simulink model "S_Tek_NDI_6DOF"  (R2025b)
settings: Solver=ode4  StartTime=0.0  StopTime=5  FixedStep=0.001  RelTol=1e-3
undefined symbols (not defined in the file): X, Y, Z
libraries: sm_lib x15, nesl_utility x13, instrumentseriallib x3, svdutilitieslib x2, sharedtransform x1, aerolibanimutils x1
(part 1 of 2)
settings Model: SimulationMode=accelerator  Creator=serha  LastModifiedBy=serha
settings OptimizationCC: DefaultParameterBehavior=Inlined  EnhancedBackFolding=on  PassReuseOutputArgsAs=Individual arguments  ZeroExternalMemoryAtStartup=off  ZeroInternalMemoryAtStartup=off  OptimizeBlockOrder=speed  DifferentSizesBufferReuse=on  EfficientTunableParamExpr=on
settings DebuggingCC: ParameterTunabilityLossMsg=error
settings SFSimCC: MATLABDynamicMemAlloc=off
settings RTWCC: SystemTargetFile=ert.tlc  GenCodeOnly=on  TemplateMakefile=ert_default_tmf  TargetLang=C++  Description=Embedded Coder
settings CodeAppCC: ForceParamTrailComments=on  IgnoreCustomStorageClasses=off  OperatorAnnotations=on  SimulinkDataObjDesc=on  SFDataObjDesc=on  InsertBlockDesc=on
settings ERTTargetCC: RootIOFormat=Structure reference  ERTCustomFileTemplate=example_file_process.tlc  TargetLangStandard=C++11 (ISO)  GenerateSampleERTMain=on  CodeInterfacePackaging=C++ class  SubcomponentCodeInterfacePackaging=C++ class

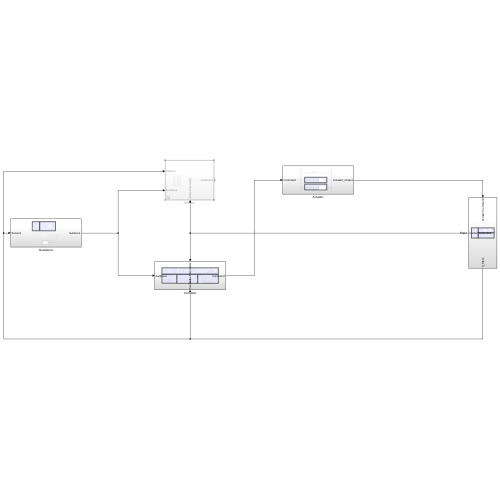
[thumbnail: Simulink's stored preview of the top-level diagram]
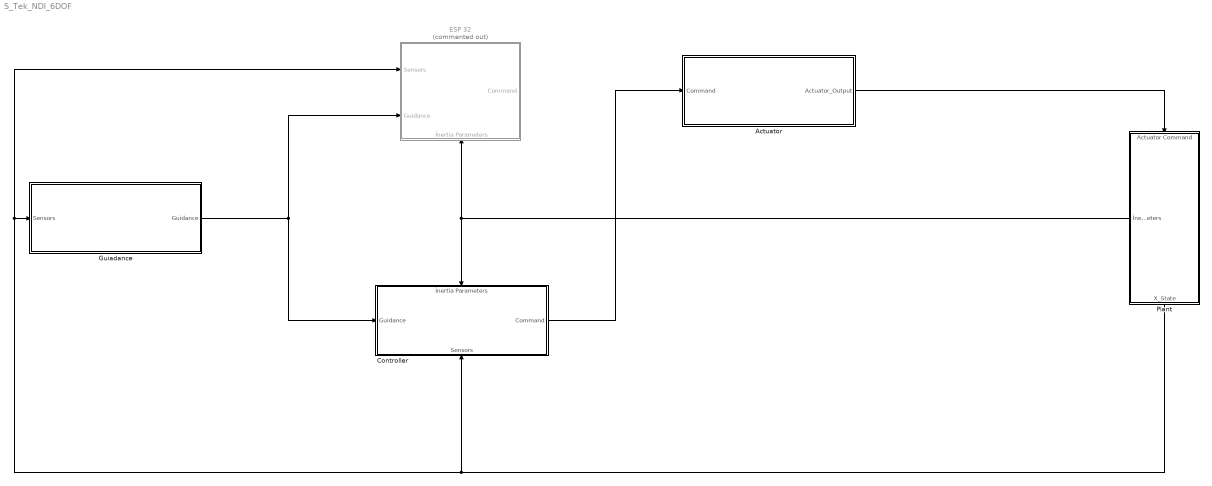
== system S_Tek_NDI_6DOF ==
  Actuator : Subsystem
  Controller : Subsystem
      settings: PortSchema="{\"entries\":[{\"content\":{\"sides\":[{\"content\":{\"connectorIds\":[\"In1\"]},\"type\":\"ConnectorPlacement.EquallySpacedRectSide\",\"uuid\":\"33b79308-0fc5-4fde-badb-0b37289253ef\"},{\"content\":{\"connectorIds\":[\"Out1\"],\"side\":\"RIGHT\"},\"type\":\"ConnectorPlacement.EquallySpacedRectSide\",\"uuid\":\"6727f24a-0c3c-4ca7-b1aa-847be9f11281\"},{\"content\":{\"connectorIds\":[\"In2\"],\"side\":\"TOP\"},\"type\":\"ConnectorPlacement.EquallySpacedRectSide\",\"uuid\":\"ebfc38b6-8c70-4d5f-9489-ae3a6562aa2e\"},{\"content\":{\"connectorIds\":[\"In3\"],\"side\":\"BOTTOM\"},\"type\":\"ConnectorPlacement.EquallySpacedRectSide\",\"uuid\":\"1b890ac9-3b95-4a4a-b282-16e3ecaf3aa4\"}]},\"type\":\"ConnectorPlacement.EquallySpacedConnector\",\"uuid\":\"d0cee92c-e3ff-4de0-b538-2dada08257b1\"}],\"packageUris\":[\"http://schema.mathworks.com/mf0/Connector/R2020b\"],\"version\":\"1.0\"}"
  ESP 32 : Subsystem  Commented=on
      settings: PortSchema="{\"entries\":[{\"content\":{\"sides\":[{\"content\":{\"connectorIds\":[\"In1\",\"In2\"]},\"type\":\"ConnectorPlacement.EquallySpacedRectSide\",\"uuid\":\"b68df156-6ec7-4598-b026-4cab0d4d3268\"},{\"content\":{\"connectorIds\":[\"Out1\"],\"side\":\"RIGHT\"},\"type\":\"ConnectorPlacement.EquallySpacedRectSide\",\"uuid\":\"75bb1db0-dca3-4be2-aa03-0ad52a7325c4\"},{\"content\":{\"side\":\"TOP\"},\"type\":\"ConnectorPlacement.EquallySpacedRectSide\",\"uuid\":\"cbcd1633-6d11-4a93-ac28-ed36ff8afac7\"},{\"content\":{\"connectorIds\":[\"In3\"],\"side\":\"BOTTOM\"},\"type\":\"ConnectorPlacement.EquallySpacedRectSide\",\"uuid\":\"f395c96f-7e1a-4722-a710-beafc27741bb\"}]},\"type\":\"ConnectorPlacement.EquallySpacedConnector\",\"uuid\":\"ea343adf-7795-4ee6-84a9-2bc60d61a1c3\"}],\"packageUris\":[\"http://schema.mathworks.com/mf0/Connector/R2020b\"],\"version\":\"1.0\"}"
  Guiadance : Subsystem
  Plant : Subsystem
      settings: PortSchema="{\"entries\":[{\"content\":{\"sides\":[{\"content\":{\"connectorIds\":[\"In1\"]},\"type\":\"ConnectorPlacement.EquallySpacedRectSide\",\"uuid\":\"29c8d766-87fc-4873-bda8-7cdfe26d04f7\"},{\"content\":{\"connectorIds\":[\"Out1\"],\"side\":\"RIGHT\"},\"type\":\"ConnectorPlacement.EquallySpacedRectSide\",\"uuid\":\"1efea905-e967-45fe-8852-2a4bff90dd9a\"},{\"content\":{\"side\":\"TOP\"},\"type\":\"ConnectorPlacement.EquallySpacedRectSide\",\"uuid\":\"b263cb17-9e53-4a4f-8000-fee4e63dac0a\"},{\"content\":{\"connectorIds\":[\"Out2\"],\"side\":\"BOTTOM\"},\"type\":\"ConnectorPlacement.EquallySpacedRectSide\",\"uuid\":\"2ade8f34-2c73-49b6-89b6-4faa6f9ebfe1\"}]},\"type\":\"ConnectorPlacement.EquallySpacedConnector\",\"uuid\":\"c146ddd7-c1b8-418c-8ccf-6973c1dcf151\"}],\"packageUris\":[\"http://schema.mathworks.com/mf0/Connector/R2020b\"],\"version\":\"1.0\"}"
  wires:
  Actuator/1(Actuator_Output) -> Plant/1(Actuator Command)
  Plant/2(İnertia Parameters) -> ESP 32/3(İnertia Parameters), Controller/2(İnertia Parameters)
  Plant/1(X_State) -> ESP 32/1(Sensors), Guiadance/1(Sensors), Controller/3(Sensors)
  Guiadance/1(Guidance) -> ESP 32/2(Guidance), Controller/1(Guidance)
  Controller/1(Command) -> Actuator/1(Command)

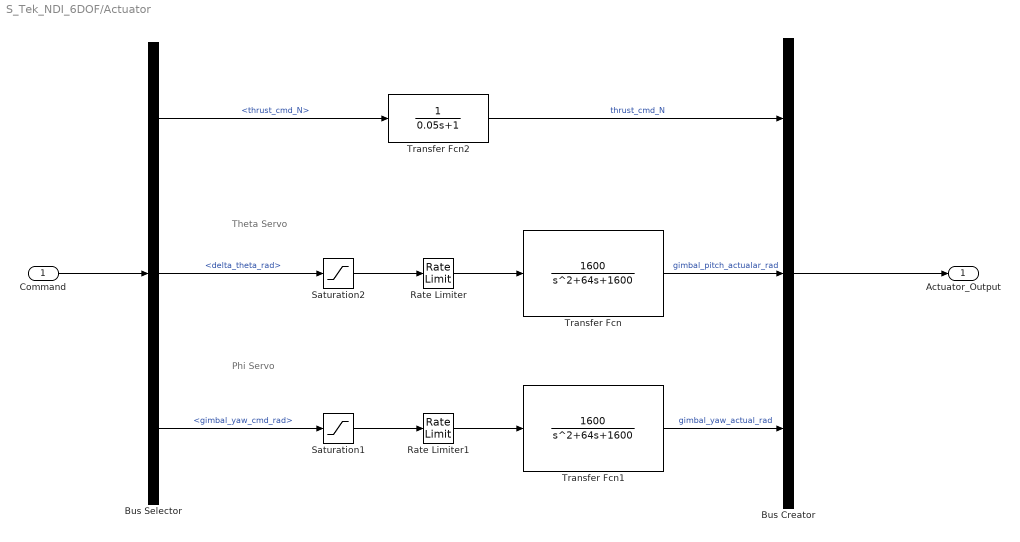
== system S_Tek_NDI_6DOF/Actuator ==
  note: Theta Servo
  note: Phi Servo
  Command : Inport
  Bus Creator : BusCreator  Inputs=3
  Bus Selector : BusSelector  OutputSignals=thrust_cmd_N,delta_theta_rad,gimbal_yaw_cmd_rad
  Rate Limiter : RateLimiter  RisingSlewLimit=deg2rad(428.5)  FallingSlewLimit=-deg2rad(428.5)  SampleTimeMode=inherited
  Rate Limiter1 : RateLimiter  RisingSlewLimit=deg2rad(428.5)  FallingSlewLimit=-deg2rad(428.5)  SampleTimeMode=inherited
  Saturation1 : Saturate  UpperLimit=deg2rad(5)  LowerLimit=-deg2rad(5)
  Saturation2 : Saturate  UpperLimit=deg2rad(5)  LowerLimit=-deg2rad(5)
  Transfer Fcn : TransferFcn  Numerator=1600  Denominator=[1 64 1600]
  Transfer Fcn1 : TransferFcn  Numerator=1600  Denominator=[1 64 1600]
  Transfer Fcn2 : TransferFcn  Denominator=[0.05 1]
  Actuator_Output : Outport
  wires:
  Bus Selector/2 -> Saturation2/1  "<delta_theta_rad>"
  Transfer Fcn/1 -> Bus Creator/2  "gimbal_pitch_actualar_rad"
  Bus Selector/1 -> Transfer Fcn2/1  "<thrust_cmd_N>"
  Command/1 -> Bus Selector/1
  Saturation1/1 -> Rate Limiter1/1
  Rate Limiter1/1 -> Transfer Fcn1/1
  Transfer Fcn1/1 -> Bus Creator/3  "gimbal_yaw_actual_rad"
  Bus Creator/1 -> Actuator_Output/1
  Saturation2/1 -> Rate Limiter/1
  Rate Limiter/1 -> Transfer Fcn/1
  Bus Selector/3 -> Saturation1/1  "<gimbal_yaw_cmd_rad>"
  Transfer Fcn2/1 -> Bus Creator/1  "thrust_cmd_N"

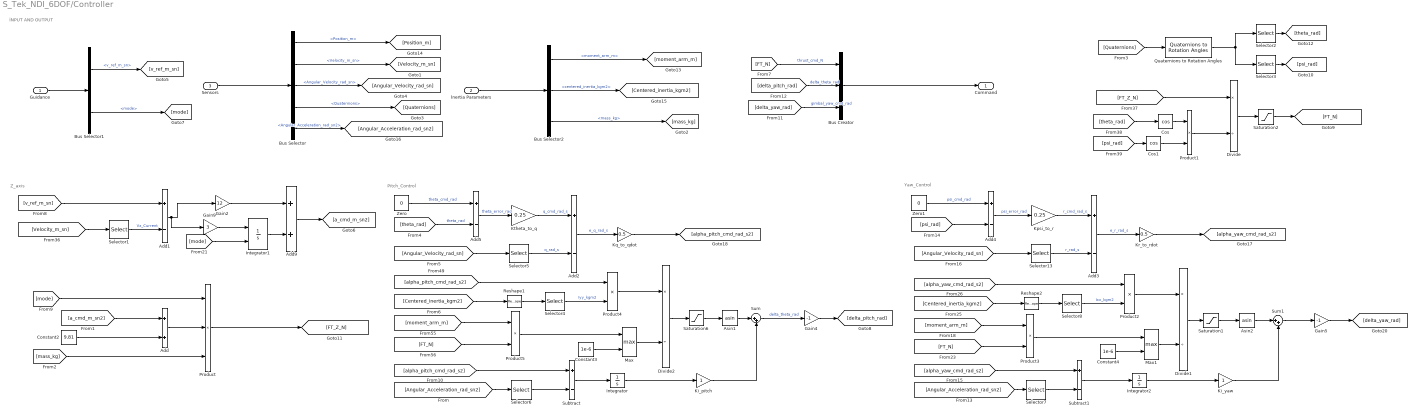
== system S_Tek_NDI_6DOF/Controller ==
  note: Z_axis
  note: Pitch_Control
  note: Yaw_Control
  note: İNPUT AND OUTPUT
  Guidance : Inport
  İnertia Parameters : Inport  Port=2
  Sensors : Inport  Port=3
  Add : Sum
  Add{1..5} (5 alike) : Sum  Inputs=+-
  Add9 : Sum
  Asin1 : Trigonometry  Operator=asin
  Asin2 : Trigonometry  Operator=asin
  Bus Creator : BusCreator  Inputs=3
  Bus Selector : BusSelector  OutputSignals=Position_m,Velocity_m_sn,Angular_Velocity_rad_sn,Quaternions,Angular_Acceleration_rad_sn2
  Bus Selector1 : BusSelector  OutputSignals=v_ref_m_sn,mode
  Bus Selector2 : BusSelector  OutputSignals=moment_arm_m,centered_inertia_kgm2,mass_kg
  Constant2 : Constant  Value=9.81
  Constant3 : Constant  Value=1e-6
  Constant4 : Constant  Value=1e-6
  Cos : Trigonometry  Operator=cos
  Cos1 : Trigonometry  Operator=cos
  Divide : Product  Inputs=*/
  Divide1 : Product  Inputs=*/
  Divide2 : Product  Inputs=*/
  Gain2 : Gain  Gain=12
  Gain4 : Gain  Gain=-1
  Gain5 : Gain  Gain=-1
  Gain9 : Gain  Gain=3
  Integrator : Integrator  LimitOutput=on  UpperSaturationLimit=5  LowerSaturationLimit=-5
  Integrator1 : Integrator  ExternalReset=rising  LimitOutput=on  UpperSaturationLimit=7.5  LowerSaturationLimit=-7.5
  Integrator2 : Integrator  LimitOutput=on  UpperSaturationLimit=5  LowerSaturationLimit=-5
  Ki_pitch : Gain
  Ki_yaw : Gain
  Kpsi_to_r : Gain  Gain=0.25
  Kq_to_qdot : Gain  Gain=0.5
  Kr_to_rdot : Gain  Gain=0.5
  Ktheta_to_q : Gain  Gain=0.25
  Max : MinMax  Function=max  Inputs=2
  Max1 : MinMax  Function=max  Inputs=2
  Product : Product  Inputs=3
  Product{1..5} (5 alike) : Product
  Quaternions to Rotation Angles : sharedtransform/Quaternions to Rotation Angles  rotationOrder=ZYX  aMode=aMode
  Reshape1 : Reshape
  Reshape2 : Reshape
  Saturation1 : Saturate  UpperLimit=1  LowerLimit=-1
  Saturation2 : Saturate  UpperLimit=600  LowerLimit=0
  Saturation6 : Saturate  UpperLimit=1  LowerLimit=-1
  Selector{1,3,7,13} (4 alike) : Selector  InputPortWidth=3  IndexOptions=Index vector (dialog)  Indices=3  OutputSizes=1
  Selector2 : Selector  InputPortWidth=3  IndexOptions=Index vector (dialog)  Indices=2  OutputSizes=1
  Selector4 : Selector  InputPortWidth=9  IndexOptions=Index vector (dialog)  Indices=5  OutputSizes=1
  Selector5 : Selector  InputPortWidth=3  IndexOptions=Index vector (dialog)  Indices=2  OutputSizes=1
  Selector6 : Selector  InputPortWidth=3  IndexOptions=Index vector (dialog)  Indices=2  OutputSizes=1
  Selector8 : Selector  InputPortWidth=9  IndexOptions=Index vector (dialog)  Indices=1  OutputSizes=1
  Subtract : Sum  Inputs=+-
  Subtract1 : Sum  Inputs=+-
  Sum : Sum  Inputs=|++
  Sum1 : Sum  Inputs=|++
  Zero : Constant  Value=0  OutDataTypeStr=Inherit: Inherit via back propagation
  Zero1 : Constant  Value=0  OutDataTypeStr=Inherit: Inherit via back propagation
  Command : Outport
  wires:
  Divide2/1 -> Saturation6/1
  Gain5/1 -> [delta_yaw_rad]
  Zero/1 -> Add5/1  "theta_cmd_rad"
  [moment_arm_m] -> Product5/1
  Gain4/1 -> [delta_pitch_rad]
  Ki_yaw/1 -> Sum1/2
  [alpha_pitch_cmd_rad_s2] -> Product4/1
  Ki_pitch/1 -> Sum/2
  Zero1/1 -> Add4/1  "psi_cmd_rad"
  Add4/1 -> Kpsi_to_r/1  "psi_error_rad"
  Product2/1 -> Divide1/1
  Subtract1/1 -> Integrator2/1
  [FT_N] -> Product3/2
  Sum/1 -> Gain4/1  "delta_theta_rad"
  Product4/1 -> Divide2/1
  Bus Selector/2 -> [Velocity_m_sn]  "<Velocity_m_sn>"
  Sum1/1 -> Gain5/1
  Constant2/1 -> Add/2
  Bus Creator/1 -> Command/1
  Selector2/1 -> [theta_rad]
  Saturation1/1 -> Asin2/1
  Asin2/1 -> Sum1/1
  [alpha_yaw_cmd_rad_s2] -> Subtract1/1
  [Velocity_m_sn] -> Selector1/1
  [delta_pitch_rad] -> Bus Creator/2  "delta_theta_rad"
  [psi_rad] -> Cos1/1
  Add2/1 -> Kq_to_qdot/1  "e_q_rad_s"
  Quaternions to Rotation Angles/1 -> Selector3/1, Selector2/1
  Selector4/1 -> Product4/2  "Iyy_kgm2"
  Selector7/1 -> Subtract1/2
  Selector1/1 -> Add1/2  "Vz_Current"
  Bus Selector2/3 -> [mass_kg]  "<mass_kg>"
  Kpsi_to_r/1 -> Add3/1  "r_cmd_rad_s"
  Add/1 -> Product/2
  Divide/1 -> Saturation2/1
  Kq_to_qdot/1 -> [alpha_pitch_cmd_rad_s2]
  Saturation2/1 -> [FT_N]
  [FT_Z_N] -> Divide/1
  [Centered_inertia_kgm2] -> Reshape2/1
  Bus Selector2/2 -> [Centered_inertia_kgm2]  "<centered_inertia_kgm2>"
  Cos1/1 -> Product1/2
  [Centered_inertia_kgm2] -> Reshape1/1
  Selector13/1 -> Add3/2  "r_rad_s"
  Max/1 -> Divide2/2
  Subtract/1 -> Integrator/1
  Reshape2/1 -> Selector8/1
  Constant3/1 -> Max/2
  Asin1/1 -> Sum/1
  Product/1 -> [FT_Z_N]
  Product5/1 -> Max/1
  Selector5/1 -> Add2/2  "q_rad_s"
  Bus Selector/3 -> [Angular_Velocity_rad_sn]  "<Angular_Velocity_rad_sn>"
  Kr_to_rdot/1 -> [alpha_yaw_cmd_rad_s2]
  [alpha_yaw_cmd_rad_s2] -> Product2/1
  Add5/1 -> Ktheta_to_q/1  "theta_error_rad"
  Constant4/1 -> Max1/2
  [mode] -> Product/1
  Max1/1 -> Divide1/2
  [moment_arm_m] -> Product3/1
  Cos/1 -> Product1/1
  Product3/1 -> Max1/1
  Bus Selector2/1 -> [moment_arm_m]  "<moment_arm_m>"
  Sensors/1 -> Bus Selector/1
  Selector6/1 -> Subtract/2
  Saturation6/1 -> Asin1/1
  [psi_rad] -> Add4/2
  [a_cmd_m_sn2] -> Add/1
  Add3/1 -> Kr_to_rdot/1  "e_r_rad_s"
  [FT_N] -> Product5/2
  Add9/1 -> [a_cmd_m_sn2]
  [mass_kg] -> Product/3
  [Quaternions] -> Quaternions to Rotation Angles/1
  Selector8/1 -> Product2/2  "Ixx_kgm2"
  Reshape1/1 -> Selector4/1
  Bus Selector/4 -> [Quaternions]  "<Quaternions>"
  Selector3/1 -> [psi_rad]
  [FT_N] -> Bus Creator/1  "thrust_cmd_N"
  Integrator/1 -> Ki_pitch/1
  [delta_yaw_rad] -> Bus Creator/3  "gimbal_yaw_cmd_rad"
  Ktheta_to_q/1 -> Add2/1  "q_cmd_rad_s"
  [alpha_pitch_cmd_rad_s2] -> Subtract/1
  İnertia Parameters/1 -> Bus Selector2/1
  Integrator2/1 -> Ki_yaw/1
  [theta_rad] -> Add5/2  "theta_rad"
  [v_ref_m_sn] -> Add1/1
  [theta_rad] -> Cos/1
  [Angular_Velocity_rad_sn] -> Selector5/1
  Divide1/1 -> Saturation1/1
  [Angular_Velocity_rad_sn] -> Selector13/1
  Product1/1 -> Divide/2
  Guidance/1 -> Bus Selector1/1
  Bus Selector1/2 -> [mode]  "<mode>"
  Bus Selector1/1 -> [v_ref_m_sn]  "<v_ref_m_sn>"
  Bus Selector/1 -> [Position_m]  "<Position_m>"
  Bus Selector/5 -> [Angular_Acceleration_rad_sn2]  "<Angular_Acceleration_rad_sn2>"
  [Angular_Acceleration_rad_sn2] -> Selector6/1
  [Angular_Acceleration_rad_sn2] -> Selector7/1
  Add1/1 -> Gain2/1, Gain9/1
  Gain2/1 -> Add9/1
  [mode] -> Integrator1/2
  Integrator1/1 -> Add9/2
  Gain9/1 -> Integrator1/1

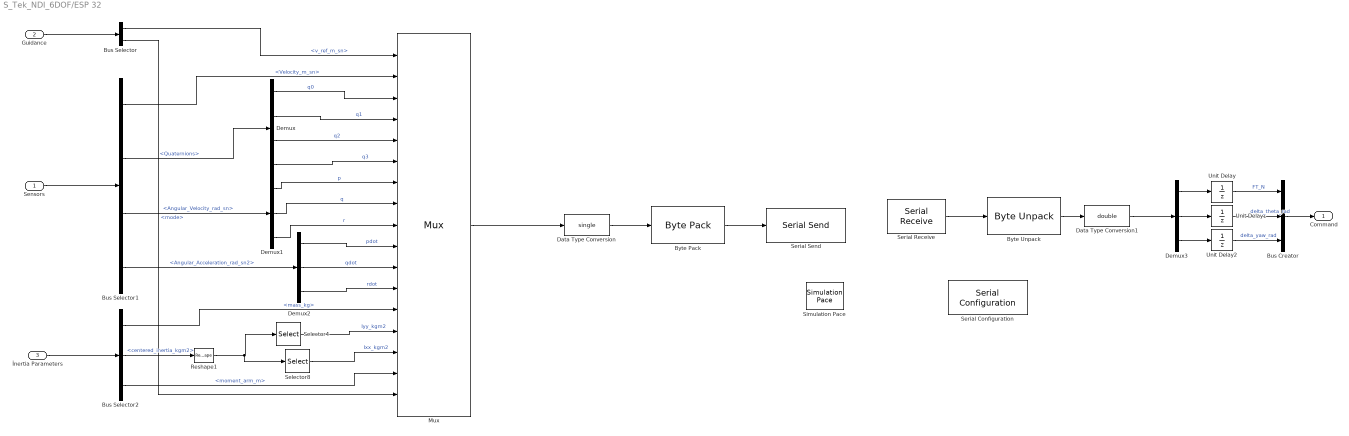
== system S_Tek_NDI_6DOF/ESP 32 ==
  Sensors : Inport
  Guidance : Inport  Port=2
  İnertia Parameters : Inport  Port=3
  Bus Creator : BusCreator  Inputs=3
  Bus Selector : BusSelector  OutputSignals=v_ref_m_sn,mode
  Bus Selector1 : BusSelector  OutputSignals=Velocity_m_sn,Quaternions,Angular_Velocity_rad_sn,Angular_Acceleration_rad_sn2
  Bus Selector2 : BusSelector  OutputSignals=mass_kg,centered_inertia_kgm2,moment_arm_m
  Byte Pack : svdutilitieslib/Byte Pack  maskPackedDataType=uint8  datatypes={'single'}  byteAlign=1  blockPlatform=arduinoert
      settings: LibrarySourceBlock=mcblib/Signal Management/Byte Pack
  Byte Unpack : svdutilitieslib/Byte Unpack  dimensions={[3 1]}  datatypes={'single'}  byteAlign=1  blockPlatform=arduinoert
      settings: LibrarySourceBlock=mcblib/Signal Management/Byte Unpack
  Data Type Conversion : DataTypeConversion  OutDataTypeStr=single  SaturateOnIntegerOverflow=off  RndMeth=Floor
  Data Type Conversion1 : DataTypeConversion  OutDataTypeStr=double  SaturateOnIntegerOverflow=off  RndMeth=Floor
  Demux : Demux
  Demux1 : Demux  Outputs=3
  Demux2 : Demux  Outputs=3
  Demux3 : Demux  Outputs=3
  Mux : Mux  Inputs=17
      settings: DisplayOption=signals
  Reshape1 : Reshape
  Selector4 : Selector  InputPortWidth=9  IndexOptions=Index vector (dialog)  Indices=5  OutputSizes=1
  Selector8 : Selector  InputPortWidth=9  IndexOptions=Index vector (dialog)  Indices=1  OutputSizes=1
  Serial Configuration : instrumentseriallib/Serial Configuration  Priority=-200000  PortSel=COM3  Port=COM3  ComPort=COM3  BaudRate=115200  DataBits=8  Parity=none  StopBits=1  ByteOrder=little-endian  FlowControl=none  Timeout=10  SimulateUsing=Interpreted execution  BlockInModel=on  aMode=1
  Serial Receive : instrumentseriallib/Serial Receive  Priority=1  PortSel=COM3  Port=COM3  ComPort=COM3  DataType=uint8  SaveDataType=uint8  ToggleHeader=off  Header=[]  ToggleDataSize=on  DataSize=12  ToggleTerminator=off  Terminator=<none>  CustomTerminator=[]  InputFormat=Column major  EnableBlockingMode=on  ActionDataUnavailable=Output last received value  ActionWhenDataUnavailable=Output last received value  CustomValue=0  SampleTime=0.001  SimulateUsing=Interpreted execution  BlockInModel=on  aMode=1  LibraryInUse=instrumentlib
  Serial Send : instrumentseriallib/Serial Send  Priority=1  PortSel=COM3  Port=COM3  ComPort=COM3  Header=[]  Terminator=<none>  CustomTerminator=[]  EnableBlockingMode=on  SimulateUsing=Interpreted execution  BlockInModel=on  aMode=1
  Simulation Pace : aerolibanimutils/Simulation Pace  SimulationPace=1  SleepMode=Auto  OutputPaceError=off  SampleTime=0.01
  Unit Delay : UnitDelay  InitialCondition=32*9.81  SampleTime=-1  HasFrameUpgradeWarning=on
  Unit Delay1 : UnitDelay  SampleTime=-1  HasFrameUpgradeWarning=on
  Unit Delay2 : UnitDelay  SampleTime=-1  HasFrameUpgradeWarning=on
  Command : Outport
  wires:
  Demux/3 -> Mux/5  "q2"
  Reshape1/1 -> Selector8/1, Selector4/1
  Bus Creator/1 -> Command/1
  Demux3/3 -> Unit Delay2/1
  Bus Selector1/1 -> Mux/2  "<Velocity_m_sn>"
  Guidance/1 -> Bus Selector/1
  Bus Selector2/2 -> Reshape1/1  "<centered_inertia_kgm2>"
  Demux3/1 -> Unit Delay/1
  Bus Selector2/3 -> Mux/16  "<moment_arm_m>"
  Data Type Conversion/1 -> Byte Pack/1
  Bus Selector1/2 -> Demux/1  "<Quaternions>"
  Bus Selector/1 -> Mux/1  "<v_ref_m_sn>"
  Bus Selector1/4 -> Demux2/1  "<Angular_Acceleration_rad_sn2>"
  Bus Selector/2 -> Mux/17  "<mode>"
  Demux3/2 -> Unit Delay1/1
  Sensors/1 -> Bus Selector1/1
  Serial Receive/1 -> Byte Unpack/1
  Byte Unpack/1 -> Data Type Conversion1/1
  Bus Selector1/3 -> Demux1/1  "<Angular_Velocity_rad_sn>"
  Selector4/1 -> Mux/14  "Iyy_kgm2"
  Demux/2 -> Mux/4  "q1"
  Demux/4 -> Mux/6  "q3"
  Mux/1 -> Data Type Conversion/1
  Demux/1 -> Mux/3  "q0"
  Demux2/3 -> Mux/12  "rdot"
  Demux1/1 -> Mux/7  "p"
  Demux1/3 -> Mux/9  "r"
  Byte Pack/1 -> Serial Send/1
  İnertia Parameters/1 -> Bus Selector2/1
  Bus Selector2/1 -> Mux/13  "<mass_kg>"
  Selector8/1 -> Mux/15  "Ixx_kgm2"
  Demux2/2 -> Mux/11  "qdot"
  Demux2/1 -> Mux/10  "pdot"
  Demux1/2 -> Mux/8  "q"
  Data Type Conversion1/1 -> Demux3/1
  Unit Delay/1 -> Bus Creator/1  "FT_N"
  Unit Delay1/1 -> Bus Creator/2  "delta_theta_rad"
  Unit Delay2/1 -> Bus Creator/3  "delta_yaw_rad"

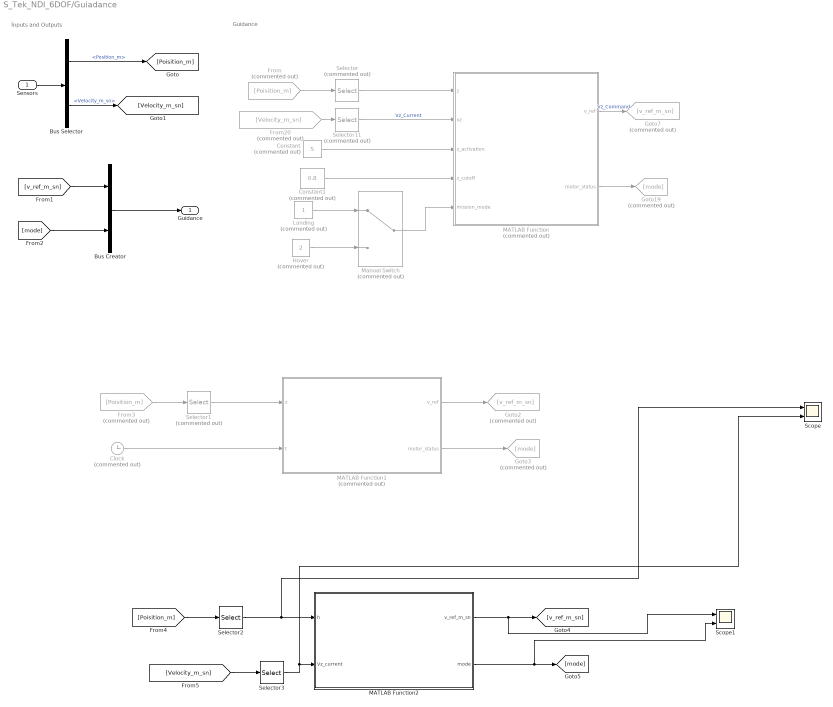
== system S_Tek_NDI_6DOF/Guiadance ==
  note: İnputs and Outputs
  note: Guidance
  Sensors : Inport
  Bus Creator : BusCreator  Inputs=2
  Bus Selector : BusSelector  OutputSignals=Position_m,Velocity_m_sn
  Clock : Clock  Commented=on
  Constant : Constant  Commented=on  Value=5
  Constant1 : Constant  Commented=on  Value=0.8
  From : From  Commented=on  GotoTag=Poisition_m
  From20 : From  Commented=on  GotoTag=Velocity_m_sn
  From3 : From  Commented=on  GotoTag=Poisition_m
  Goto19 : Goto  Commented=on  GotoTag=mode
  Goto2 : Goto  Commented=on  GotoTag=v_ref_m_sn
  Goto3 : Goto  Commented=on  GotoTag=mode
  Goto7 : Goto  Commented=on  GotoTag=v_ref_m_sn
  Hover : Constant  Commented=on  Value=2
  Landing : Constant  Commented=on
  MATLAB Function : MATLAB Function  Commented=on  TreatAsAtomicUnit=on
  MATLAB Function1 : MATLAB Function  Commented=on  TreatAsAtomicUnit=on
  MATLAB Function2 : MATLAB Function  TreatAsAtomicUnit=on
  Manual Switch : ManualSwitch  Commented=on
  Scope : Scope  NumInputPorts=2
      settings: ActiveDisplayYMinimum=0.3729081547310884  ActiveDisplayYMaximum=11.069676871696545
  Scope1 : Scope  NumInputPorts=2
      settings: ActiveDisplayYMinimum=-1  ActiveDisplayYMaximum=1
  Selector : Selector  Commented=on  InputPortWidth=3  IndexOptions=Index vector (dialog)  Indices=3  OutputSizes=1
  Selector1 : Selector  Commented=on  InputPortWidth=3  IndexOptions=Index vector (dialog)  Indices=3  OutputSizes=1
  Selector11 : Selector  Commented=on  InputPortWidth=3  IndexOptions=Index vector (dialog)  Indices=3  OutputSizes=1
  Selector2 : Selector  InputPortWidth=3  IndexOptions=Index vector (dialog)  Indices=3  OutputSizes=1
  Selector3 : Selector  InputPortWidth=3  IndexOptions=Index vector (dialog)  Indices=3  OutputSizes=1
  Guidance : Outport
  wires:
  Constant/1 -> MATLAB Function/3(z_activation)
  MATLAB Function/2(motor_status) -> Goto19/1
  Hover/1 -> Manual Switch/2
  From/1 -> Selector/1
  Manual Switch/1 -> MATLAB Function/5(mission_mode)
  Constant1/1 -> MATLAB Function/4(z_cutoff)
  Landing/1 -> Manual Switch/1
  Selector/1 -> MATLAB Function/1(z)
  Selector11/1 -> MATLAB Function/2(vz)  "Vz_Current"
  MATLAB Function/1(v_ref) -> Goto7/1  "Vz_Command"
  From20/1 -> Selector11/1
  Bus Creator/1 -> Guidance/1
  [v_ref_m_sn] -> Bus Creator/1
  [mode] -> Bus Creator/2
  Sensors/1 -> Bus Selector/1
  Bus Selector/2 -> [Velocity_m_sn]  "<Velocity_m_sn>"
  Bus Selector/1 -> [Poisition_m]  "<Position_m>"
  From3/1 -> Selector1/1
  Selector1/1 -> MATLAB Function1/1(z)
  MATLAB Function1/1(v_ref) -> Goto2/1
  MATLAB Function1/2(motor_status) -> Goto3/1
  Clock/1 -> MATLAB Function1/2(t)
  MATLAB Function2/2(mode) -> Scope1/2, [mode]
  MATLAB Function2/1(v_ref_m_sn) -> Scope1/1, [v_ref_m_sn]
  Selector2/1 -> Scope/1, MATLAB Function2/1(h)
  [Poisition_m] -> Selector2/1
  [Velocity_m_sn] -> Selector3/1
  Selector3/1 -> Scope/2, MATLAB Function2/2(Vz_current)

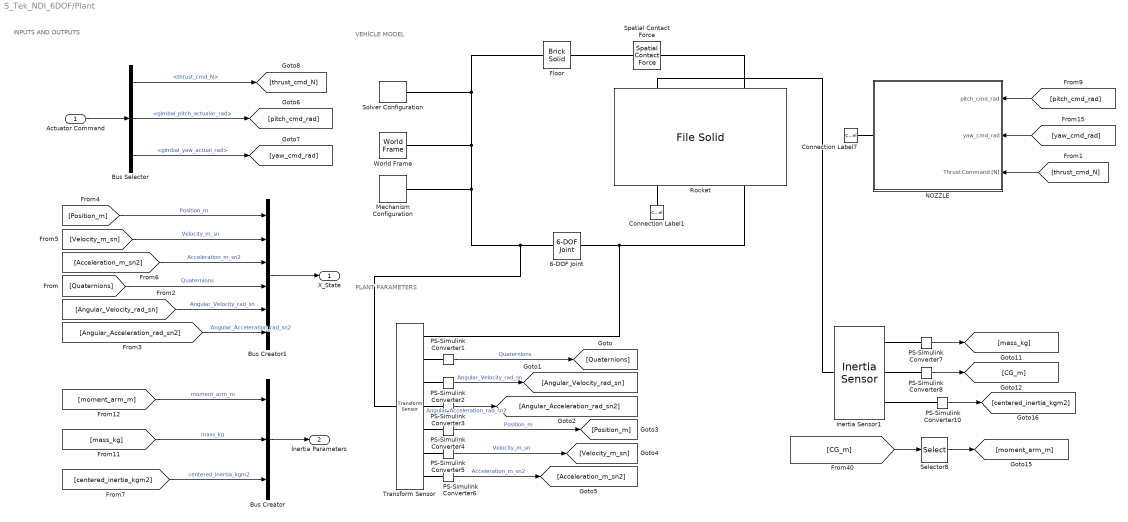
== system S_Tek_NDI_6DOF/Plant ==
  note: iNPUTS AND OUTPUTS
  note: VEHİCLE MODEL
  note: PLANT PARAMETERS
  Actuator Command : Inport
  6-DOF Joint : sm_lib/Joints/6-DOF Joint  JointMode=Normal  CompositeWrenchDir=FollowerOnBase  CompositeWrenchFrame=BaseFrame  SenseConstraintForce=off  SenseConstraintTorque=off  SenseTotalForce=off  SenseTotalTorque=off  PxPositionTargetSpecify=off  PxPositionTargetPriority=High  PxPositionTargetValue=0  PxPositionTargetValueUnits=m  PxVelocityTargetSpecify=off  PxVelocityTargetPriority=High  PxVelocityTargetValue=0  PxVelocityTargetValueUnits=m/s  PxEquilibriumPosition=0  PxEquilibriumPositionUnits=m  PxSpringStiffness=0  PxSpringStiffnessUnits=N/m  PxDampingCoefficient=0  PxDampingCoefficientUnits=N/(m/s)  PxLowerLimitSpecify=off  PxLowerLimitBound=-1  PxLowerLimitBoundUnits=m  PxLowerLimitStiffness=1e6  PxLowerLimitStiffnessUnits=N/m  PxLowerLimitDamping=1e3  PxLowerLimitDampingUnits=N/(m/s)  PxLowerLimitTransitionRegionWidth=1e-4  PxLowerLimitTransitionRegionWidthUnits=m  PxUpperLimitSpecify=off  PxUpperLimitBound=1  PxUpperLimitBoundUnits=m  PxUpperLimitStiffness=1e6  PxUpperLimitStiffnessUnits=N/m  PxUpperLimitDamping=1e3  PxUpperLimitDampingUnits=N/(m/s)  PxUpperLimitTransitionRegionWidth=1e-4  PxUpperLimitTransitionRegionWidthUnits=m  PxTorqueActuationMode=NoTorque  PxMotionActuationMode=ComputedMotion  PxSensePosition=off  PxSenseVelocity=off  PxSenseAcceleration=off  PxSenseTorqueForce=off  PxSenseLowerLimitTorqueForce=off  PxSenseUpperLimitTorqueForce=off  PyPositionTargetSpecify=off  PyPositionTargetPriority=High  PyPositionTargetValue=0  PyPositionTargetValueUnits=m  PyVelocityTargetSpecify=off  PyVelocityTargetPriority=High  PyVelocityTargetValue=0  PyVelocityTargetValueUnits=m/s  PyEquilibriumPosition=0  PyEquilibriumPositionUnits=m  PySpringStiffness=0  PySpringStiffnessUnits=N/m  PyDampingCoefficient=0  PyDampingCoefficientUnits=N/(m/s)  PyLowerLimitSpecify=off  PyLowerLimitBound=-1  PyLowerLimitBoundUnits=m  PyLowerLimitStiffness=1e6  PyLowerLimitStiffnessUnits=N/m  PyLowerLimitDamping=1e3  PyLowerLimitDampingUnits=N/(m/s)  PyLowerLimitTransitionRegionWidth=1e-4  PyLowerLimitTransitionRegionWidthUnits=m  PyUpperLimitSpecify=off  PyUpperLimitBound=1  PyUpperLimitBoundUnits=m  PyUpperLimitStiffness=1e6  PyUpperLimitStiffnessUnits=N/m  PyUpperLimitDamping=1e3  PyUpperLimitDampingUnits=N/(m/s)  PyUpperLimitTransitionRegionWidth=1e-4  PyUpperLimitTransitionRegionWidthUnits=m  PyTorqueActuationMode=NoTorque  PyMotionActuationMode=ComputedMotion  PySensePosition=off  PySenseVelocity=off  PySenseAcceleration=off  PySenseTorqueForce=off  PySenseLowerLimitTorqueForce=off  PySenseUpperLimitTorqueForce=off  PzPositionTargetSpecify=on  PzPositionTargetPriority=High  PzPositionTargetValue=10  PzPositionTargetValueUnits=m  PzVelocityTargetSpecify=off  PzVelocityTargetPriority=High  PzVelocityTargetValue=0  PzVelocityTargetValueUnits=m/s  PzEquilibriumPosition=0  PzEquilibriumPositionUnits=m  PzSpringStiffness=0  PzSpringStiffnessUnits=N/m  PzDampingCoefficient=0  PzDampingCoefficientUnits=N/(m/s)  PzLowerLimitSpecify=off  PzLowerLimitBound=-1  PzLowerLimitBoundUnits=m  PzLowerLimitStiffness=1e6  PzLowerLimitStiffnessUnits=N/m  PzLowerLimitDamping=1e3  PzLowerLimitDampingUnits=N/(m/s)  PzLowerLimitTransitionRegionWidth=1e-4  PzLowerLimitTransitionRegionWidthUnits=m  PzUpperLimitSpecify=off  PzUpperLimitBound=1  PzUpperLimitBoundUnits=m  PzUpperLimitStiffness=1e6  PzUpperLimitStiffnessUnits=N/m  PzUpperLimitDamping=1e3  PzUpperLimitDampingUnits=N/(m/s)  PzUpperLimitTransitionRegionWidth=1e-4  PzUpperLimitTransitionRegionWidthUnits=m  PzTorqueActuationMode=NoTorque  PzMotionActuationMode=ComputedMotion  PzSensePosition=off  PzSenseVelocity=off  PzSenseAcceleration=off  PzSenseTorqueForce=off  PzSenseLowerLimitTorqueForce=off  PzSenseUpperLimitTorqueForce=off  SphPositionTargetSpecify=off  SphPositionTargetPriority=High  SphPositionTargetRotationMethod=StandardAxis  SphPositionTargetFollAlignAxisA=+X  SphPositionTargetBaseAlignAxisA=+Y  SphPositionTargetFollAlignAxisB=+Y  SphPositionTargetBaseAlignAxisB=+Z  SphPositionTargetRotationStandardAxis=+X  SphPositionTargetRotationAngle=10  SphPositionTargetRotationAngleUnits=deg  SphPositionTargetRotationArbitraryAxis=[0 0 1]  SphPositionTargetRotationSequenceAxes=FollowerAxes  SphPositionTargetRotationSequence=ZYX  SphPositionTargetRotationSequenceAngles=[0 0 0]  SphPositionTargetRotationSequenceAnglesUnits=deg  SphPositionTargetRotationMatrix=[1 0 0;0 1 0;0 0 1]  SphPositionTargetQuaternion=[1 0 0 0]  SphVelocityTargetSpecify=off  SphVelocityTargetPriority=High  SphVelocityTargetValue=[0 0 0]  SphVelocityTargetValueUnits=deg/s  SphVelocityTargetInFollowerFrame=on  SphEqPosRotationMethod=None  SphEqPosFollAlignAxisA=+X  SphEqPosBaseAlignAxisA=+Y  SphEqPosFollAlignAxisB=+Y  SphEqPosBaseAlignAxisB=+Z  SphEqPosRotationStandardAxis=+Z  SphEqPosRotationAngle=0  SphEqPosRotationAngleUnits=deg  SphEqPosRotationArbitraryAxis=[0 0 1]  SphEqPosRotationSequenceAxes=FollowerAxes  SphEqPosRotationSequence=XYX  SphEqPosRotationSequenceAngles=[0 0 0]  SphEqPosRotationSequenceAnglesUnits=deg  SphEqPosRotationMatrix=[1 0 0;0 1 0;0 0 1]  SphEqPosQuaternion=[1 0 0 0]  SphSpringStiffness=0  SphSpringStiffnessUnits=N*m/deg  SphDampingCoefficient=0  SphDampingCoefficientUnits=N*m/(deg/s)  SphLowerLimitSpecify=off  SphLowerLimitBound=15  SphLowerLimitBoundUnits=deg  SphLowerLimitStiffness=1e4  SphLowerLimitStiffnessUnits=N*m/deg  SphLowerLimitDamping=10  SphLowerLimitDampingUnits=N*m/(deg/s)  SphLowerLimitTransitionRegionWidth=0.1  SphLowerLimitTransitionRegionWidthUnits=deg  SphUpperLimitSpecify=off  SphUpperLimitBound=45  SphUpperLimitBoundUnits=deg  SphUpperLimitStiffness=1e4  SphUpperLimitStiffnessUnits=N*m/deg  SphUpperLimitDamping=10  SphUpperLimitDampingUnits=N*m/(deg/s)  SphUpperLimitTransitionRegionWidth=0.1  SphUpperLimitTransitionRegionWidthUnits=deg  SphTorqueActuationMode=NoTorque  SphActuateTorqueX=off  SphActuateTorqueY=off  SphActuateTorqueZ=off  SphActuateTorque=off  SphActuationFrame=BaseFrame  SphSensePosition=off  SphSenseVelocityX=off  SphSenseVelocityY=off  SphSenseVelocityZ=off  SphSenseVelocity=off  SphSenseAccelerationX=off  SphSenseAccelerationY=off  SphSenseAccelerationZ=off  SphSenseAcceleration=off  SphSenseLowerLimitTorqueMag=off  SphSenseUpperLimitTorqueMag=off  SphSensingFrame=BaseFrame
  Bus Creator : BusCreator  Inputs=3
  Bus Creator1 : BusCreator  Inputs=6
  Bus Selector : BusSelector  OutputSignals=thrust_cmd_N,gimbal_pitch_actualar_rad,gimbal_yaw_actual_rad
  Connection Label1 : ConnectionLabel  Label=NOZZLE
  Connection Label7 : ConnectionLabel  Label=NOZZLE
  Floor : sm_lib/Body Elements/Brick Solid  BrickDimensions=[5 5 0.5]  BrickDimensionsUnits=m  ExportEntireGeometry=on  InertiaType=CalculateFromGeometry  BasedOnType=Density  Density=0  DensityUnits=kg/m^3  Mass=1  MassUnits=kg  CenterOfMass=[0 0 0]  CenterOfMassUnits=m  MomentsOfInertia=[1 1 1]  MomentsOfInertiaUnits=kg*m^2  ProductsOfInertia=[0 0 0]  ProductsOfInertiaUnits=kg*m^2  GraphicType=FromGeometry  MarkerShape=Sphere  MarkerSize=10  GraphicVisPropType=SimpleVisualProperties  GraphicDiffuseColor=[1 0.6667 0]  GraphicOpacity=1  GraphicSpecularColor=[0.5 0.5 0.5 1.0]  GraphicAmbientColor=[0.15 0.15 0.15 1.0]  GraphicEmissiveColor=[0.0 0.0 0.0 1.0]  GraphicShininess=75  DoExposeReferenceFrame=on  SerializedFrames=<Frames/>
  Inertia Sensor1 : sm_lib/Body Elements/Inertia Sensor  SensorExtent=Mechanism  SpanWeldJoints=off  ExcludeGroundedBodies=off  MeasurementFrame=Attached  SenseMass=on  SenseCenterOfMass=on  SenseInertiaMatrix=off  SenseCenteredInertiaMatrix=on  SensePrincipalInertiaMatrix=off  SenseRotationMatrix=off  GraphicType=PrincipalInertiaFrame  PrincipalInertiaFrameSize=20  GraphicVisPropType=SimpleVisualProperties  GraphicDiffuseColor=[0.5 0.5 0.5]  GraphicOpacity=1  GraphicSpecularColor=[0.5 0.5 0.5 1.0]  GraphicAmbientColor=[0.15 0.15 0.15 1.0]  GraphicEmissiveColor=[0.0 0.0 0.0 1.0]  GraphicShininess=75
  Mechanism Configuration : sm_lib/Utilities/Mechanism Configuration  UniformGravity=Constant  GravityVector=[0 0 -9.80665]  GravityVectorUnits=m/s^2  LinearizationDelta=0.001  JointModeTransitionNonlinearIterations=2
  NOZZLE : Subsystem
  PS-Simulink Converter{1..8,10} (9 alike) : nesl_utility/PS-Simulink Converter  PhysicalDomain=network_engine_domain  SubClassName=ps_output  LeftPortType=input  RightPortType=output  PseudoPeriodic=off  Frequencies=[]  VectorFormat=inherit  Unit=inherit  AffineConversion=off
  Rocket : sm_lib/Body Elements/File Solid  ExtGeomFileName=C:\Users\serha\Desktop\protopitop.STEP  UnitType=Custom  ExtGeomFileUnits=cm  StepReaderType=HEX  ExportConvexHullGeometry=on  InertiaType=CalculateFromGeometry  BasedOnType=Mass  Density=1000  DensityUnits=kg/m^3  Mass=31  MassUnits=kg  CenterOfMass=[0 0 0]  CenterOfMassUnits=m  MomentsOfInertia=[1 1 1]  MomentsOfInertiaUnits=kg*m^2  ProductsOfInertia=[0 0 0]  ProductsOfInertiaUnits=kg*m^2  GraphicType=FromGeometry  MarkerShape=Sphere  MarkerSize=10  GraphicVisPropType=SimpleVisualProperties  GraphicDiffuseColor=[0.5 0.5 0.5]  GraphicOpacity=1  GraphicSpecularColor=[0.5 0.5 0.5 1.0]  GraphicAmbientColor=[0.15 0.15 0.15 1.0]  GraphicEmissiveColor=[0.0 0.0 0.0 1.0]  GraphicShininess=75  DoExposeReferenceFrame=off  SerializedFrames=<Frames><Frame><Id>Frame2</Id><Value><Name>TVC</Name><Origin><Source>GeometricFeature</Source><FeatureName>point 7</FeatureName></Origin><PrimaryAxis><DefinedDirection>+Z</DefinedDirection><Source>ReferenceFrame</Source><SourceDirection>+X</SourceDirection><FeatureName></FeatureName></PrimaryAxis><SecondaryAxis><DefinedDirection>+X</DefinedDirection><Source>ReferenceFrame</Source><SourceDirection>-Z</SourceDirection><FeatureName></FeatureName></SecondaryAxis></Value></Frame><Frame><Id>Frame3</Id><Value><Name>İnertia_Sensor</Name><Origin><Source>GeometricFeature</Source><FeatureName>point 7</FeatureName></Origin><PrimaryAxis><DefinedDirection>+Z</DefinedDirection><Source>ReferenceFrame</Source><SourceDirection>+Z</SourceDirection><FeatureName></FeatureName></PrimaryAxis><SecondaryAxis><DefinedDirection>+X</DefinedDirection><Source>ReferenceFrame</Source><SourceDirection>+X</SourceDirection><FeatureName></FeatureName></SecondaryAxis></Value></Frame><Frame><Id>Frame4</Id><Value><Name>Sensors</Name><Origin><Source>GeometricFeature</Source><FeatureName>planar surface 1</FeatureName></Origin><PrimaryAxis><DefinedDirection>+Z</DefinedDirection><Source>ReferenceFrame</Source><SourceDirection>+Z</SourceDirection><FeatureName></FeatureName></PrimaryAxis><SecondaryAxis><DefinedDirection>+X</DefinedDirection><Source>ReferenceFrame</Source><SourceDirection>+X</SourceDirection><FeatureName></FeatureName></SecondaryAxis></Value></Frame></Frames>
  Selector8 : Selector  InputPortWidth=3  IndexOptions=Index vector (dialog)  Indices=3  OutputSizes=1
  Solver Configuration : nesl_utility/Solver Configuration  PhysicalDomain=network_engine_domain  SubClassName=solver  LeftPortType=input  RightPortType=generic  Tones=[]  Harmonics=[]  SimulateNoise=off  Profile=off  UseLocalSampling=off  EnableSwitchedLinearOptims=on  FrequencyDomain=off  UseCCode=off  RelTol=0.001  AbsTol=1e-06  MinStep=1e-09  ToWorkspace=off  RevertToSquareIcSolve=off  NumHomotopyIterations=100  PhasorMode=off  PhasorModeNumHarmonics=1  ConsistencySolver=NEWTON_XTOL_AFTER_FTOL  IndexReductionMethod=DerivativeReplacement  DoDC=off  ResidualTolerance=1e-09  ConsistencyTolSource=GLOBAL  ConsistencyAbsTol=0.001  ConsistencyRelTol=0.001  ConsistencyTolFactor=0.001  UseLocalSolver=on  LocalSolverChoice=NE_BACKWARD_EULER_ADVANCER  ResolveIndetEquations=on  FunctionEvalNumThread=1  LocalSolverSampleTime=0.001  DoFixedCost=off  MaxNonlinIter=3  MaxModeIter=2  ComputeImpulses=off  ImpulseIterations=2  LinearAlgebra=Sparse  LinearAlgebraNumThread=0  EquationFormulation=NE_TIME_EF  DelaysMemoryBudget=1024  AutomaticFiltering=on  FilteringTimeConstant=0.001  PartitionStorageMethod=AS_NEEDED  PartitionMemoryBudget=1024  PartitionMethod=FAST  MultibodyUseLocalSolver=off  MultibodyLocalSolverChoice=ODE1  MultibodyLocalSolverSampleTime=0.001
  Spatial Contact Force : sm_lib/Forces and Torques/Spatial Contact Force  SenseSeparationDistance=off  NormalForceType=SmoothSpringDamper  NormalStiffness=1e6  NormalStiffnessUnits=N/m  NormalDamping=1e3  NormalDampingUnits=N/(m/s)  NormalTransitionRegionWidth=1e-4  NormalTransitionRegionWidthUnits=m  FrictionType=SmoothStickSlip  CoefficientOfStaticFriction=0.5  CoefficientOfDynamicFriction=0.3  FrictionalCriticalVelocity=1e-3  FrictionalCriticalVelocityUnits=m/s  SenseContactSignal=off  SensePenetrationDepth=off  SenseNormalVelocity=off  SenseTangentialVelocity=off  SensingForceTorqueDirection=BaseOnFollower  SensingForceTorqueResolutionFrame=ContactFrame  SenseNormalForce=off  SenseNormalForceMagnitude=off  SenseNormalTorque=off  SenseFrictionalForce=off  SenseFrictionalForceMagnitude=off  SenseFrictionalTorque=off  SenseTotalForce=off  SenseTotalTorque=off  SenseContactBaseRotation=off  SenseContactBaseTranslation=off  SenseContactFollowerRotation=off  SenseContactFollowerTranslation=off  ZeroCrossDetectContactStartAndEnd=off
  Transform Sensor : sm_lib/Frames and Transforms/Transform Sensor  MeasurementFrame=World  RotationSequence=ZYX  SenseAngle=off  SenseAxis=off  SenseQ=on  SenseR=off  SenseRotationSequence=off  SenseOmegaX=off  SenseOmegaY=off  SenseOmegaZ=off  SenseOmega=on  SenseQDot=off  SenseRDot=off  SenseRotationSequenceDot=off  SenseAlphaX=off  SenseAlphaY=off  SenseAlphaZ=off  SenseAlpha=on  SenseQDDot=off  SenseRDDot=off  SenseX=off  SenseY=off  SenseZ=off  SenseXYZ=on  SenseRad=off  SenseAzim=off  SenseDist=off  SenseInc=off  SenseXDot=off  SenseYDot=off  SenseZDot=off  SenseXYZDot=on  SenseRadDot=off  SenseAzimDot=off  SenseDistDot=off  SenseIncDot=off  SenseXDDot=off  SenseYDDot=off  SenseZDDot=off  SenseXYZDDot=on  SenseRadDDot=off  SenseAzimDDot=off  SenseDistDDot=off  SenseIncDDot=off
  World Frame : sm_lib/Frames and Transforms/World Frame
  X_State : Outport
  İnertia Parameters : Outport  Port=2
  wires:
  Bus Creator/1 -> İnertia Parameters/1
  PS-Simulink Converter2/1 -> [Angular_Velocity_rad_sn]  "Angular_Velocity_rad_sn"
  PS-Simulink Converter8/1 -> [CG_m]
  Bus Selector/3 -> [yaw_cmd_rad]  "<gimbal_yaw_actual_rad>"
  [Angular_Acceleration_rad_sn2] -> Bus Creator1/6  "Angular_Acceleration_rad_sn2"
  [yaw_cmd_rad] -> NOZZLE/2(yaw_cmd_rad)
  [Acceleration_m_sn2] -> Bus Creator1/3  "Acceleration_m_sn2"
  Bus Selector/2 -> [pitch_cmd_rad]  "<gimbal_pitch_actualar_rad>"
  [Quaternions] -> Bus Creator1/4  "Quaternions"
  PS-Simulink Converter3/1 -> [Angular_Acceleration_rad_sn2]  "Angular_Acceleration_rad_sn2"
  PS-Simulink Converter10/1 -> [centered_inertia_kgm2]
  Selector8/1 -> [moment_arm_m]
  PS-Simulink Converter1/1 -> [Quaternions]  "Quaternions"
  Actuator Command/1 -> Bus Selector/1
  [mass_kg] -> Bus Creator/2  "mass_kg"
  [Position_m] -> Bus Creator1/1  "Position_m"
  [moment_arm_m] -> Bus Creator/1  "moment_arm_m"
  Bus Creator1/1 -> X_State/1
  PS-Simulink Converter7/1 -> [mass_kg]
  [thrust_cmd_N] -> NOZZLE/3(Thrust Command [N])
  PS-Simulink Converter5/1 -> [Velocity_m_sn]  "Velocity_m_sn"
  [Angular_Velocity_rad_sn] -> Bus Creator1/5  "Angular_Velocity_rad_sn"
  Bus Selector/1 -> [thrust_cmd_N]  "<thrust_cmd_N>"
  [centered_inertia_kgm2] -> Bus Creator/3  "centered_inertia_kgm2"
  PS-Simulink Converter6/1 -> [Acceleration_m_sn2]  "Acceleration_m_sn2"
  [CG_m] -> Selector8/1
  [pitch_cmd_rad] -> NOZZLE/1("pitch_cmd_rad ")
  [Velocity_m_sn] -> Bus Creator1/2  "Velocity_m_sn"
  PS-Simulink Converter4/1 -> [Position_m]  "Position_m"
  connections:
  Solver Configuration/RConn1 -- World Frame/RConn1 -- Transform Sensor/LConn1 -- 6-DOF Joint/LConn1 -- Mechanism Configuration/RConn1 -- Floor/RConn1
  Transform Sensor/RConn1 -- Rocket/LConn2 -- 6-DOF Joint/RConn1
  Transform Sensor/RConn6 -- PS-Simulink Converter5/LConn1
  NOZZLE/RConn1 -- Connection Label7/LConn1
  PS-Simulink Converter2/LConn1 -- Transform Sensor/RConn3
  Connection Label1/LConn1 -- Rocket/LConn1
  Floor/LConn1 -- Spatial Contact Force/LConn1
  PS-Simulink Converter3/LConn1 -- Transform Sensor/RConn4
  PS-Simulink Converter1/LConn1 -- Transform Sensor/RConn2
  Rocket/RConn2 -- Spatial Contact Force/RConn1
  PS-Simulink Converter7/LConn1 -- Inertia Sensor1/RConn1
  Inertia Sensor1/RConn2 -- PS-Simulink Converter8/LConn1
  PS-Simulink Converter4/LConn1 -- Transform Sensor/RConn5
  Rocket/RConn1 -- Inertia Sensor1/LConn1
  Transform Sensor/RConn7 -- PS-Simulink Converter6/LConn1
  Inertia Sensor1/RConn3 -- PS-Simulink Converter10/LConn1

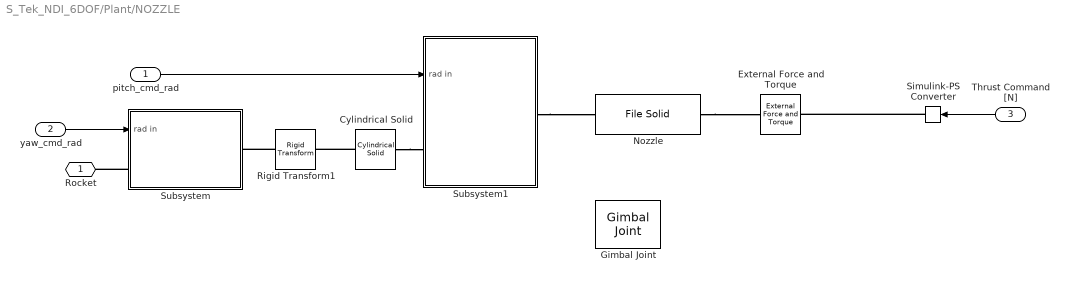
== system S_Tek_NDI_6DOF/Plant/NOZZLE ==
  "pitch_cmd_rad " : Inport
  yaw_cmd_rad : Inport  Port=2
  Thrust Command [N] : Inport  Port=3
  Cylindrical Solid : sm_lib/Body Elements/Cylindrical Solid  CylinderRadius=0.05  CylinderRadiusUnits=m  CylinderLength=0.02  CylinderLengthUnits=m  ExportEntireGeometry=off  InertiaType=CalculateFromGeometry  BasedOnType=Mass  Density=1000  DensityUnits=kg/m^3  Mass=0.01  MassUnits=kg  CenterOfMass=[0 0 0]  CenterOfMassUnits=m  MomentsOfInertia=[1 1 1]  MomentsOfInertiaUnits=kg*m^2  ProductsOfInertia=[0 0 0]  ProductsOfInertiaUnits=kg*m^2  GraphicType=FromGeometry  MarkerShape=Sphere  MarkerSize=10  GraphicVisPropType=SimpleVisualProperties  GraphicDiffuseColor=[0.5 0.5 0.5]  GraphicOpacity=1  GraphicSpecularColor=[0.5 0.5 0.5 1.0]  GraphicAmbientColor=[0.15 0.15 0.15 1.0]  GraphicEmissiveColor=[0.0 0.0 0.0 1.0]  GraphicShininess=75  DoExposeReferenceFrame=on  SerializedFrames=|
      | <Frames>
      | 
      |   <Frame>
      |     <Id>Frame1</Id>
      |     <Value>
      |       <Name>F1</Name>
      |       <Origin>
      |         <Source>ReferenceFrame</Source>
      |         <FeatureName></FeatureName>
      |       </Origin>
      |       <PrimaryAxis>
      |         <DefinedDirection>+Z</DefinedDirection>
      |         <Source>ReferenceFrame</Source>
      |         <SourceDirection>+Z</SourceDirection>
      |         <FeatureName></FeatureName>
      |       </PrimaryAxis>
      |       <SecondaryAxis>
      |         <DefinedDirection>+X</DefinedDirection>
      |         <Source>ReferenceFrame</Source>
      |         <SourceDirection>+X</SourceDirection>
      |         <FeatureName></FeatureName>
      |       </SecondaryAxis>
      |     </Value>
      |   </Frame>
      | 
      | </Frames>
  External Force and Torque : sm_lib/Forces and Torques/External Force and Torque  EnableForceX=off  EnableForceY=off  EnableForceZ=on  EnableForce=off  ForceResolutionFrame=AttachedFrame  EnableTorqueX=off  EnableTorqueY=off  EnableTorqueZ=off  EnableTorque=off  TorqueResolutionFrame=AttachedFrame
  Gimbal Joint : sm_lib/Joints/Gimbal Joint  JointMode=Normal  CompositeWrenchDir=FollowerOnBase  CompositeWrenchFrame=BaseFrame  SenseConstraintForce=off  SenseConstraintTorque=off  SenseTotalForce=off  SenseTotalTorque=off  RxPositionTargetSpecify=off  RxPositionTargetPriority=High  RxPositionTargetValue=0  RxPositionTargetValueUnits=deg  RxVelocityTargetSpecify=off  RxVelocityTargetPriority=High  RxVelocityTargetValue=0  RxVelocityTargetValueUnits=deg/s  RxEquilibriumPosition=0  RxEquilibriumPositionUnits=deg  RxSpringStiffness=0  RxSpringStiffnessUnits=N*m/deg  RxDampingCoefficient=0  RxDampingCoefficientUnits=N*m/(deg/s)  RxLowerLimitSpecify=off  RxLowerLimitBound=-90  RxLowerLimitBoundUnits=deg  RxLowerLimitStiffness=1e4  RxLowerLimitStiffnessUnits=N*m/deg  RxLowerLimitDamping=10  RxLowerLimitDampingUnits=N*m/(deg/s)  RxLowerLimitTransitionRegionWidth=0.1  RxLowerLimitTransitionRegionWidthUnits=deg  RxUpperLimitSpecify=off  RxUpperLimitBound=90  RxUpperLimitBoundUnits=deg  RxUpperLimitStiffness=1e4  RxUpperLimitStiffnessUnits=N*m/deg  RxUpperLimitDamping=10  RxUpperLimitDampingUnits=N*m/(deg/s)  RxUpperLimitTransitionRegionWidth=0.1  RxUpperLimitTransitionRegionWidthUnits=deg  RxTorqueActuationMode=NoTorque  RxMotionActuationMode=ComputedMotion  RxSensePosition=off  RxSenseVelocity=off  RxSenseAcceleration=off  RxSenseTorqueForce=off  RxSenseLowerLimitTorqueForce=off  RxSenseUpperLimitTorqueForce=off  RyPositionTargetSpecify=off  RyPositionTargetPriority=High  RyPositionTargetValue=0  RyPositionTargetValueUnits=deg  RyVelocityTargetSpecify=off  RyVelocityTargetPriority=High  RyVelocityTargetValue=0  RyVelocityTargetValueUnits=deg/s  RyEquilibriumPosition=0  RyEquilibriumPositionUnits=deg  RySpringStiffness=0  RySpringStiffnessUnits=N*m/deg  RyDampingCoefficient=0  RyDampingCoefficientUnits=N*m/(deg/s)  RyLowerLimitSpecify=off  RyLowerLimitBound=-90  RyLowerLimitBoundUnits=deg  RyLowerLimitStiffness=1e4  RyLowerLimitStiffnessUnits=N*m/deg  RyLowerLimitDamping=10  RyLowerLimitDampingUnits=N*m/(deg/s)  RyLowerLimitTransitionRegionWidth=0.1  RyLowerLimitTransitionRegionWidthUnits=deg  RyUpperLimitSpecify=off  RyUpperLimitBound=90  RyUpperLimitBoundUnits=deg  RyUpperLimitStiffness=1e4  RyUpperLimitStiffnessUnits=N*m/deg  RyUpperLimitDamping=10  RyUpperLimitDampingUnits=N*m/(deg/s)  RyUpperLimitTransitionRegionWidth=0.1  RyUpperLimitTransitionRegionWidthUnits=deg  RyTorqueActuationMode=NoTorque  RyMotionActuationMode=ComputedMotion  RySensePosition=off  RySenseVelocity=off  RySenseAcceleration=off  RySenseTorqueForce=off  RySenseLowerLimitTorqueForce=off  RySenseUpperLimitTorqueForce=off  RzPositionTargetSpecify=off  RzPositionTargetPriority=High  RzPositionTargetValue=0  RzPositionTargetValueUnits=deg  RzVelocityTargetSpecify=off  RzVelocityTargetPriority=High  RzVelocityTargetValue=0  RzVelocityTargetValueUnits=deg/s  RzEquilibriumPosition=0  RzEquilibriumPositionUnits=deg  RzSpringStiffness=0  RzSpringStiffnessUnits=N*m/deg  RzDampingCoefficient=0  RzDampingCoefficientUnits=N*m/(deg/s)  RzLowerLimitSpecify=off  RzLowerLimitBound=-90  RzLowerLimitBoundUnits=deg  RzLowerLimitStiffness=1e4  RzLowerLimitStiffnessUnits=N*m/deg  RzLowerLimitDamping=10  RzLowerLimitDampingUnits=N*m/(deg/s)  RzLowerLimitTransitionRegionWidth=0.1  RzLowerLimitTransitionRegionWidthUnits=deg  RzUpperLimitSpecify=off  RzUpperLimitBound=90  RzUpperLimitBoundUnits=deg  RzUpperLimitStiffness=1e4  RzUpperLimitStiffnessUnits=N*m/deg  RzUpperLimitDamping=10  RzUpperLimitDampingUnits=N*m/(deg/s)  RzUpperLimitTransitionRegionWidth=0.1  RzUpperLimitTransitionRegionWidthUnits=deg  RzTorqueActuationMode=NoTorque  RzMotionActuationMode=ComputedMotion  RzSensePosition=off  RzSenseVelocity=off  RzSenseAcceleration=off  RzSenseTorqueForce=off  RzSenseLowerLimitTorqueForce=off  RzSenseUpperLimitTorqueForce=off
  Nozzle : sm_lib/Body Elements/File Solid  ExtGeomFileName=C:\Users\serha\Desktop\nozll.STEP  UnitType=FromFile  ExtGeomFileUnits=m  StepReaderType=HEX  ExportConvexHullGeometry=off  InertiaType=CalculateFromGeometry  BasedOnType=Mass  Density=1000  DensityUnits=kg/m^3  Mass=1  MassUnits=kg  CenterOfMass=[0 0 0]  CenterOfMassUnits=m  MomentsOfInertia=[1 1 1]  MomentsOfInertiaUnits=kg*m^2  ProductsOfInertia=[0 0 0]  ProductsOfInertiaUnits=kg*m^2  GraphicType=FromGeometry  MarkerShape=Sphere  MarkerSize=10  GraphicVisPropType=SimpleVisualProperties  GraphicDiffuseColor=[0.5 0.5 0.5]  GraphicOpacity=1  GraphicSpecularColor=[0.5 0.5 0.5 1.0]  GraphicAmbientColor=[0.15 0.15 0.15 1.0]  GraphicEmissiveColor=[0.0 0.0 0.0 1.0]  GraphicShininess=75  DoExposeReferenceFrame=off  SerializedFrames=<Frames><Frame><Id>Frame1</Id><Value><Name>Rocket</Name><Origin><Source>GeometricFeature</Source><FeatureName>planar surface 1</FeatureName></Origin><PrimaryAxis><DefinedDirection>+Z</DefinedDirection><Source>ReferenceFrame</Source><SourceDirection>+Y</SourceDirection><FeatureName></FeatureName></PrimaryAxis><SecondaryAxis><DefinedDirection>-Y</DefinedDirection><Source>ReferenceFrame</Source><SourceDirection>+X</SourceDirection><FeatureName></FeatureName></SecondaryAxis></Value></Frame><Frame><Id>Frame2</Id><Value><Name>Thrust</Name><Origin><Source>GeometricFeature</Source><FeatureName>planar surface 3</FeatureName></Origin><PrimaryAxis><DefinedDirection>+Z</DefinedDirection><Source>ReferenceFrame</Source><SourceDirection>+Z</SourceDirection><FeatureName></FeatureName></PrimaryAxis><SecondaryAxis><DefinedDirection>+X</DefinedDirection><Source>ReferenceFrame</Source><SourceDirection>+X</SourceDirection><FeatureName></FeatureName></SecondaryAxis></Value></Frame></Frames>
  Rigid Transform1 : sm_lib/Frames and Transforms/Rigid Transform  RotationMethod=StandardAxis  FollAlignAxisA=+X  BaseAlignAxisA=+Y  FollAlignAxisB=+Y  BaseAlignAxisB=+Z  RotationStandardAxis=+X  RotationAngle=-90  RotationAngleUnits=deg  RotationArbitraryAxis=[0 0 1]  RotationSequenceAxes=FollowerAxes  RotationSequence=XYX  RotationSequenceAngles=[0 0 0]  RotationSequenceAnglesUnits=deg  RotationMatrix=[1 0 0;0 1 0;0 0 1]  Quaternion=[1 0 0 0]  TranslationMethod=None  TranslationCartesianOffset=[0 0 0]  TranslationCartesianOffsetUnits=m  TranslationStandardAxis=+Z  TranslationStandardOffset=0  TranslationStandardOffsetUnits=m  TranslationROffset=0  TranslationROffsetUnits=m  TranslationThetaOffset=0  TranslationThetaOffsetUnits=deg  TranslationZOffset=0  TranslationZOffsetUnits=m
  Simulink-PS Converter : nesl_utility/Simulink-PS Converter  PhysicalDomain=network_engine_domain  SubClassName=ps_input  LeftPortType=input  RightPortType=output  PseudoPeriodic=off  Frequencies=[]  NoiseDistribution=none  NoiseParameters=[]  Unit=1  AffineConversion=off  FilteringAndDerivatives=filter  SimscapeFilterOrder=1  InputFilterTimeConstant=0.001  UdotUserProvided=0
  Subsystem : Subsystem
  Subsystem1 : Subsystem
  Rocket : PMIOPort  Side=Right
  wires:
  yaw_cmd_rad/1 -> Subsystem/1(rad in)
  Thrust Command [N]/1 -> Simulink-PS Converter/1
  "pitch_cmd_rad "/1 -> Subsystem1/1(rad in)
  connections:
  Rigid Transform1/LConn1 -- Subsystem/RConn1
  Subsystem/LConn1 -- Rocket/RConn1
  Nozzle/RConn1 -- External Force and Torque/RConn1
  Simulink-PS Converter/RConn1 -- External Force and Torque/LConn1
  Subsystem1/RConn1 -- Nozzle/LConn1
  Cylindrical Solid/RConn1 -- Rigid Transform1/RConn1
  Cylindrical Solid/LConn1 -- Subsystem1/LConn1

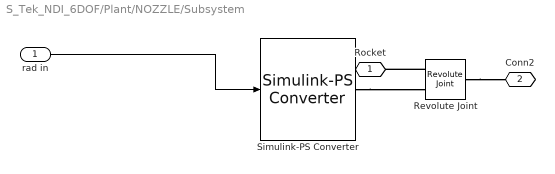
== system S_Tek_NDI_6DOF/Plant/NOZZLE/Subsystem ==
  rad in : Inport
  Revolute Joint : sm_lib/Joints/Revolute Joint  JointMode=Normal  CompositeWrenchDir=FollowerOnBase  CompositeWrenchFrame=BaseFrame  SenseConstraintForce=off  SenseConstraintTorque=off  SenseTotalForce=off  SenseTotalTorque=off  PositionTargetSpecify=off  PositionTargetPriority=High  PositionTargetValue=0  PositionTargetValueUnits=deg  VelocityTargetSpecify=off  VelocityTargetPriority=High  VelocityTargetValue=0  VelocityTargetValueUnits=deg/s  EquilibriumPosition=0  EquilibriumPositionUnits=deg  SpringStiffness=0  SpringStiffnessUnits=N*m/deg  DampingCoefficient=0  DampingCoefficientUnits=N*m/(deg/s)  LowerLimitSpecify=off  LowerLimitBound=-90  LowerLimitBoundUnits=deg  LowerLimitStiffness=1e4  LowerLimitStiffnessUnits=N*m/deg  LowerLimitDamping=10  LowerLimitDampingUnits=N*m/(deg/s)  LowerLimitTransitionRegionWidth=0.1  LowerLimitTransitionRegionWidthUnits=deg  UpperLimitSpecify=off  UpperLimitBound=90  UpperLimitBoundUnits=deg  UpperLimitStiffness=1e4  UpperLimitStiffnessUnits=N*m/deg  UpperLimitDamping=10  UpperLimitDampingUnits=N*m/(deg/s)  UpperLimitTransitionRegionWidth=0.1  UpperLimitTransitionRegionWidthUnits=deg  TorqueActuationMode=ComputedTorque  MotionActuationMode=InputMotion  SensePosition=off  SenseVelocity=off  SenseAcceleration=off  SenseTorqueForce=off  SenseLowerLimitTorqueForce=off  SenseUpperLimitTorqueForce=off
  Simulink-PS Converter : nesl_utility/Simulink-PS Converter  PhysicalDomain=network_engine_domain  SubClassName=ps_input  LeftPortType=input  RightPortType=output  PseudoPeriodic=off  Frequencies=[]  NoiseDistribution=none  NoiseParameters=[]  Unit=1  AffineConversion=off  FilteringAndDerivatives=filter  SimscapeFilterOrder=2  InputFilterTimeConstant=0.001  UdotUserProvided=2
  Rocket : PMIOPort  Side=Left
  Conn2 : PMIOPort  Port=2  Side=Right
  wires:
  rad in/1 -> Simulink-PS Converter/1
  connections:
  Revolute Joint/RConn1 -- Conn2/RConn1
  Revolute Joint/LConn1 -- Rocket/RConn1
  Simulink-PS Converter/RConn1 -- Revolute Joint/LConn2
